simulink model "F16"  (R2024b)
settings: Solver=VariableStepAuto  StartTime=0  StopTime=Tend  RelTol=1e-3
values from neighbouring files (symbols this model uses):
  Param = load_F16_params()    [F16AeroFM.m]    (also in runF16.m; test_with_julia.m; trim_and_linearize.m)
libraries: aerolibasang x3, shared6dof x1, aerolibatmos2 x1
settings Model: Creator=sherpa  LastModifiedBy=sherpa
settings SolverCC: AlgebraicLoopSolver=TrustRegion
settings DataIOCC: SaveFormat=StructureWithTime
settings OptimizationCC: BlockReduction=off  DefaultParameterBehavior=Inlined  OptimizeBlockIOStorage=off  BufferReuse=off
settings DebuggingCC: AlgebraicLoopMsg=none  InitInArrayFormatMsg=none
settings ModelReferenceCC: EnableRefExpFcnMdlSchedulingChecks=on
settings RTWCC: GPUComputeCapability=3.5  DLArmComputeVersion=19.05

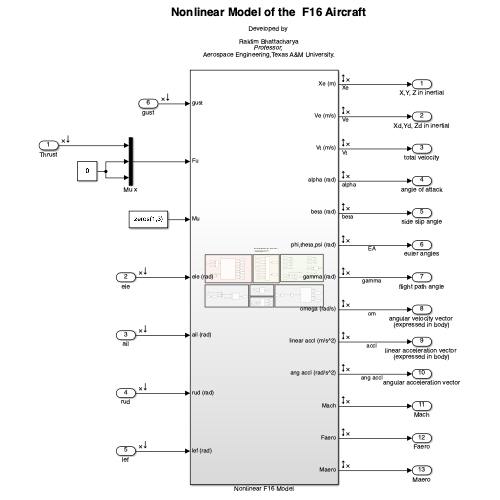
[thumbnail: Simulink's stored preview of the top-level diagram]
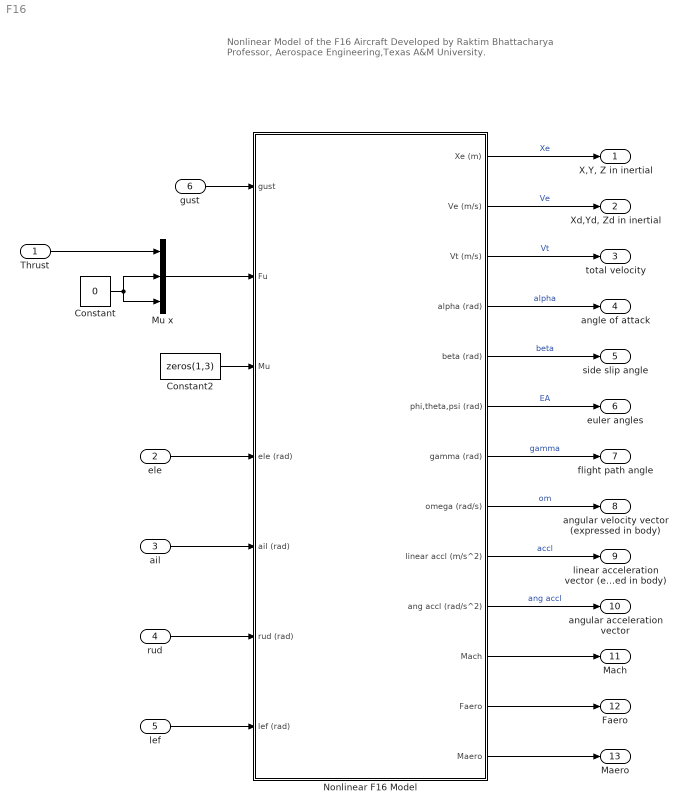
== system F16 ==
  note: Nonlinear Model of the F16 Aircraft
      |
      | Developed by
      |
      | Raktim Bhattacharya
      | Professor,
      | Aerospace Engineering,Texas A&M University.
  Thrust : Inport
  ele : Inport  Port=2
  ail : Inport  Port=3
  rud : Inport  Port=4
  lef : Inport  Port=5
  gust : Inport  Port=6
  Constant : Constant  Value=0
  Constant2 : Constant  Value=zeros(1,3)
  Mu x : Mux  Inputs=3
  Nonlinear F16 Model : Subsystem
  "X,Y, Z in inertial" : Outport
  "Xd,Yd, Zd in inertial" : Outport  Port=2
  total velocity : Outport  Port=3
  angle of attack : Outport  Port=4
  side slip angle : Outport  Port=5
  euler angles : Outport  Port=6
  flight path angle : Outport  Port=7
  angular velocity vector (expressed in body) : Outport  Port=8
  linear acceleration vector (expressed in body) : Outport  Port=9
  angular acceleration vector : Outport  Port=10
  Mach : Outport  Port=11
  Faero : Outport  Port=12
  Maero : Outport  Port=13
  wires:
  Nonlinear F16 Model/1(Xe (m)) -> "X,Y, Z in inertial"/1  "Xe"
  Nonlinear F16 Model/3(Vt (m/s)) -> total velocity/1  "Vt"
  Nonlinear F16 Model/4(alpha (rad)) -> angle of attack/1  "alpha"
  Nonlinear F16 Model/5(beta (rad)) -> side slip angle/1  "beta"
  Nonlinear F16 Model/7(gamma (rad)) -> flight path angle/1  "gamma"
  Nonlinear F16 Model/8(omega (rad/s)) -> angular velocity vector (expressed in body)/1  "om"
  Nonlinear F16 Model/9(linear accl (m/s^2)) -> linear acceleration vector (expressed in body)/1  "accl"
  Nonlinear F16 Model/6(phi,theta,psi (rad)) -> euler angles/1  "EA"
  Nonlinear F16 Model/2(Ve (m/s)) -> "Xd,Yd, Zd in inertial"/1  "Ve"
  Nonlinear F16 Model/10(ang accl (rad/s^2)) -> angular acceleration vector/1  "ang accl"
  Nonlinear F16 Model/11(Mach) -> Mach/1
  Constant2/1 -> Nonlinear F16 Model/3(Mu)
  Thrust/1 -> Mu x/1
  Constant/1 -> Mu x/3, Mu x/2
  Mu x/1 -> Nonlinear F16 Model/2(Fu)
  ele/1 -> Nonlinear F16 Model/4(ele (rad))
  rud/1 -> Nonlinear F16 Model/6(rud (rad))
  lef/1 -> Nonlinear F16 Model/7(lef (rad))
  ail/1 -> Nonlinear F16 Model/5(ail (rad))
  gust/1 -> Nonlinear F16 Model/1(gust)
  Nonlinear F16 Model/12(Faero) -> Faero/1
  Nonlinear F16 Model/13(Maero) -> Maero/1

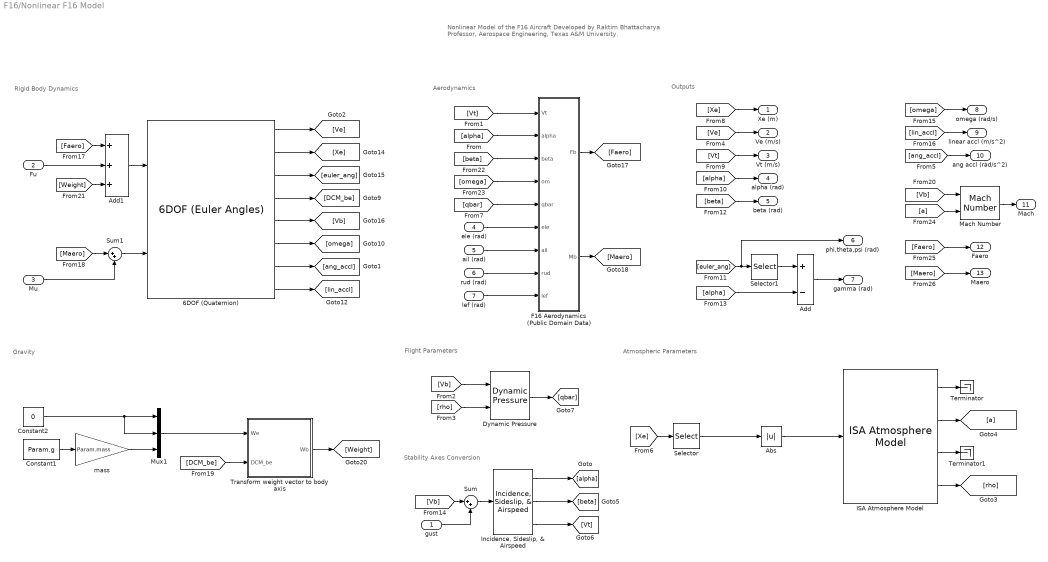
== system F16/Nonlinear F16 Model ==
  note: Gravity
  note: Nonlinear Model of the F16 Aircraft
      |
      | Developed by Raktim Bhattacharya
      | Professor, Aerospace Engineering,
      | Texas A&M University.
  note: Aerodynamics
  note: Outputs
  note: Rigid Body Dynamics
  note: Stability Axes Conversion
  note: Atmospheric Parameters
  note: Flight Parameters
  gust : Inport  PortDimensions=3
  Fu : Inport  Port=2  PortDimensions=3
  Mu : Inport  Port=3  PortDimensions=3
  ele (rad) : Inport  Port=4
  ail (rad) : Inport  Port=5
  rud (rad) : Inport  Port=6
  lef (rad) : Inport  Port=7
  6DOF (Quaternion) : shared6dof/6DOF (Euler Angles)  units=Metric (MKS)  mtype=Fixed  rep=Euler Angles  xme_0=IC.inertial_position  Vm_0=IC.body_velocity  eul_0=IC.euler_angles  pm_0=IC.omega  mass_0=Param.mass  mass_e=0.5  mass_f=2.0  inertia=Param.moi  inertia_e=eye(3)  inertia_f=2*eye(3)  k_quat=1.0  vre_flag=on  abi_flag=off  aMode=0  xme_statename={'Xe', 'Ye', 'Ze'}  Vm_statename={'U', 'v', 'w'}  eul_statename=''  quat_statename={'qr', 'qi', 'qj', 'qk'}  pm_statename={'p', 'q', 'r'}  mass_statename=''
      settings: LibrarySourceBlock=aerolib6dof2/6DOF (Quaternion)
  Abs : Abs  SaturateOnIntegerOverflow=off
  Add : Sum  Inputs=+-
  Add1 : Sum  Inputs=+++
  Constant1 : Constant  Value=Param.g
  Constant2 : Constant  Value=0
  Dynamic Pressure : aerolibasang/Dynamic Pressure
  F16 Aerodynamics (Public Domain Data) : Subsystem
  ISA Atmosphere Model : aerolibatmos2/ISA Atmosphere Model  useExtended=off  action=Warning  custom=off  viscosityOut=off  g=9.80665  gamma=1.4  R=287.0531  L=0.0065  h_trop=11000  h_strat=20000  rho0=1.225  P0=101325  T0=288.15  h0=0  S=110.4  Tref=273.15  muref=1.716e-5
  "Incidence, Sideslip, & Airspeed" : aerolibasang/Incidence, Sideslip, & Airspeed
  Mach Number : aerolibasang/Mach Number
  Mux1 : Mux  Inputs=3
  Selector : Selector  InputPortWidth=3  IndexOptions=Index vector (dialog)  Indices=3  OutputSizes=1
  Selector1 : Selector  InputPortWidth=3  IndexOptions=Index vector (dialog)  Indices=2  OutputSizes=1
  Sum : Sum  Inputs=|++
  Sum1 : Sum  Inputs=|++
  Terminator : Terminator
  Terminator1 : Terminator
  Transform weight vector to body axis : MATLAB Function  TreatAsAtomicUnit=on
  mass : Gain  Gain=Param.mass
  Xe (m) : Outport
  Ve (m/s) : Outport  Port=2
  Vt (m/s) : Outport  Port=3
  alpha (rad) : Outport  Port=4
  beta (rad) : Outport  Port=5
  phi,theta,psi (rad) : Outport  Port=6
  gamma (rad) : Outport  Port=7
  omega (rad/s) : Outport  Port=8
  linear accl (m/s^2) : Outport  Port=9
  ang accl (rad/s^2) : Outport  Port=10
  Mach : Outport  Port=11
  Faero : Outport  Port=12
  Maero : Outport  Port=13
  wires:
  [Xe] -> Selector/1
  [beta] -> beta (rad)/1
  "Incidence, Sideslip, & Airspeed"/3 -> [Vt]
  ISA Atmosphere Model/3 -> Terminator1/1
  ISA Atmosphere Model/1 -> Terminator/1
  ISA Atmosphere Model/4 -> [rho]
  [rho] -> Dynamic Pressure/2
  [lin_accl] -> linear accl (m/s^2)/1
  [alpha] -> alpha (rad)/1
  ISA Atmosphere Model/2 -> [a]
  [Vb] -> Dynamic Pressure/1
  Add/1 -> gamma (rad)/1
  [Vt] -> Vt (m/s)/1
  "Incidence, Sideslip, & Airspeed"/2 -> [beta]
  Selector1/1 -> Add/1
  "Incidence, Sideslip, & Airspeed"/1 -> [alpha]
  Selector/1 -> Abs/1
  [alpha] -> Add/2
  [euler_ang] -> phi,theta,psi (rad)/1, Selector1/1
  [omega] -> omega (rad/s)/1
  Dynamic Pressure/1 -> [qbar]
  [Xe] -> Xe (m)/1
  Constant1/1 -> mass/1
  mass/1 -> Mux1/3
  Mux1/1 -> Transform weight vector to body axis/1(We)
  Transform weight vector to body axis/1(Wb) -> [Weight]
  [DCM_be] -> Transform weight vector to body axis/2(DCM_be)
  Constant2/1 -> Mux1/2, Mux1/1
  [Faero] -> Add1/1
  Fu/1 -> Add1/2
  [Weight] -> Add1/3
  Add1/1 -> 6DOF (Quaternion)/1
  [Vb] -> Sum/1
  Sum/1 -> "Incidence, Sideslip, & Airspeed"/1
  gust/1 -> Sum/2
  [Maero] -> Sum1/1
  Mu/1 -> Sum1/2
  6DOF (Quaternion)/1 -> [Ve]
  6DOF (Quaternion)/2 -> [Xe]
  6DOF (Quaternion)/3 -> [euler_ang]
  6DOF (Quaternion)/4 -> [DCM_be]
  6DOF (Quaternion)/5 -> [Vb]
  6DOF (Quaternion)/6 -> [omega]
  6DOF (Quaternion)/7 -> [ang_accl]
  6DOF (Quaternion)/8 -> [lin_accl]
  [Ve] -> Ve (m/s)/1
  [ang_accl] -> ang accl (rad/s^2)/1
  [Vb] -> Mach Number/1
  [a] -> Mach Number/2
  Mach Number/1 -> Mach/1
  F16 Aerodynamics (Public Domain Data)/1(Fb) -> [Faero]
  Sum1/1 -> 6DOF (Quaternion)/2
  F16 Aerodynamics (Public Domain Data)/2(Mb) -> [Maero]
  [Vt] -> F16 Aerodynamics (Public Domain Data)/1(Vt)
  [alpha] -> F16 Aerodynamics (Public Domain Data)/2(alpha)
  [beta] -> F16 Aerodynamics (Public Domain Data)/3(beta)
  [omega] -> F16 Aerodynamics (Public Domain Data)/4(om)
  [qbar] -> F16 Aerodynamics (Public Domain Data)/5(qbar)
  ele (rad)/1 -> F16 Aerodynamics (Public Domain Data)/6(ele)
  ail (rad)/1 -> F16 Aerodynamics (Public Domain Data)/7(ail)
  rud (rad)/1 -> F16 Aerodynamics (Public Domain Data)/8(rud)
  lef (rad)/1 -> F16 Aerodynamics (Public Domain Data)/9(lef)
  Abs/1 -> ISA Atmosphere Model/1
  [Faero] -> Faero/1
  [Maero] -> Maero/1

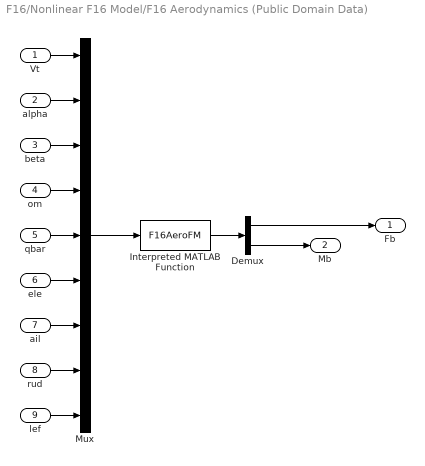
== system F16/Nonlinear F16 Model/F16 Aerodynamics (Public Domain Data) ==
  Vt : Inport
  alpha : Inport  Port=2
  beta : Inport  Port=3
  om : Inport  Port=4
  qbar : Inport  Port=5
  ele : Inport  Port=6
  ail : Inport  Port=7
  rud : Inport  Port=8
  lef : Inport  Port=9
  Demux : Demux  Outputs=2
  Interpreted MATLAB Function : MATLABFcn  MATLABFcn=F16AeroFM  OutputDimensions=6
  Mux : Mux  Inputs=9
  Fb : Outport  PortDimensions=3
  Mb : Outport  Port=2  PortDimensions=3
  wires:
  om/1 -> Mux/4
  beta/1 -> Mux/3
  qbar/1 -> Mux/5
  alpha/1 -> Mux/2
  ele/1 -> Mux/6
  Vt/1 -> Mux/1
  ail/1 -> Mux/7
  rud/1 -> Mux/8
  lef/1 -> Mux/9
  Mux/1 -> Interpreted MATLAB Function/1
  Demux/1 -> Fb/1
  Demux/2 -> Mb/1
  Interpreted MATLAB Function/1 -> Demux/1

== matlab function F16/Nonlinear F16 Model/Transform weight vector to body axis ==
  data: We input; Wb output; DCM_be input
function Wb = fcn(We,DCM_be)
Wb = DCM_be*We; % Weight in body coordinate system. DCM_be is correct, no need for transpose. They must have fixed it in this version.
